simulink model "CMOS_Differential_Stage"
settings: Solver=ode23t  StopTime=0.005  MaxStep=1e-6  RelTol=1e-5  AbsTol=1e-6
undefined symbols (not defined in the file or in its folder): CMOSParams
libraries: fl_lib x18, nesl_utility x9, simulink x2
settings Model: Creator=Final Year B.Tech ECE Project Team  LastModifiedBy=Antigravity MATLAB Automation

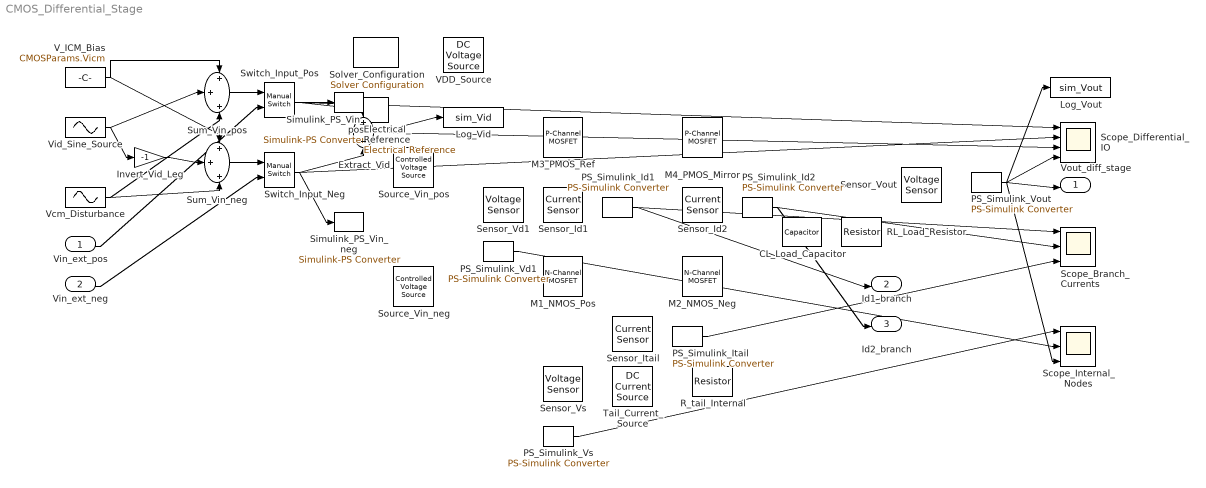
== system CMOS_Differential_Stage ==
  V_ICM_Bias : Constant  Value=CMOSParams.Vicm
  Vid_Sine_Source : Sin  Amplitude=CMOSParams.trans_Vid_peak / 2  Frequency=2*pi*CMOSParams.trans_freq
  Invert_Vid_Leg : Gain  Gain=-1
  Vcm_Disturbance : Sin  Amplitude=CMOSParams.cm_test_amp  Frequency=2*pi*CMOSParams.cm_test_freq
  Sum_Vin_pos : Sum  Inputs=+++
  Sum_Vin_neg : Sum  Inputs=+++
  Vin_ext_pos : Inport  Port=1
  Vin_ext_neg : Inport  Port=2
  Switch_Input_Pos : simulink/Signal Routing/Manual Switch
  Switch_Input_Neg : simulink/Signal Routing/Manual Switch
  Solver_Configuration : nesl_utility/Solver Configuration
  Electrical_Reference : fl_lib/Electrical/Electrical Elements/Electrical Reference
  VDD_Source : fl_lib/Electrical/Electrical Sources/DC Voltage Source  v0=CMOSParams.Vdd
  Simulink_PS_Vin_pos : nesl_utility/Simulink-PS Converter
  Source_Vin_pos : fl_lib/Electrical/Electrical Sources/Controlled Voltage Source
  Simulink_PS_Vin_neg : nesl_utility/Simulink-PS Converter
  Source_Vin_neg : fl_lib/Electrical/Electrical Sources/Controlled Voltage Source
  M1_NMOS_Pos : fl_lib/Electrical/Electrical Elements/N-Channel MOSFET  vth=CMOSParams.nmos.Vth  kp=CMOSParams.nmos.Kp  lambda=CMOSParams.nmos.lambda  rd=CMOSParams.nmos.rd  rs=CMOSParams.nmos.rs
  M2_NMOS_Neg : fl_lib/Electrical/Electrical Elements/N-Channel MOSFET  vth=CMOSParams.nmos.Vth  kp=CMOSParams.nmos.Kp  lambda=CMOSParams.nmos.lambda  rd=CMOSParams.nmos.rd  rs=CMOSParams.nmos.rs
  M3_PMOS_Ref : fl_lib/Electrical/Electrical Elements/P-Channel MOSFET  vth=CMOSParams.pmos.Vth_mag  kp=CMOSParams.pmos.Kp  lambda=CMOSParams.pmos.lambda  rd=CMOSParams.pmos.rd  rs=CMOSParams.pmos.rs
  M4_PMOS_Mirror : fl_lib/Electrical/Electrical Elements/P-Channel MOSFET  vth=CMOSParams.pmos.Vth_mag  kp=CMOSParams.pmos.Kp  lambda=CMOSParams.pmos.lambda  rd=CMOSParams.pmos.rd  rs=CMOSParams.pmos.rs
  Tail_Current_Source : fl_lib/Electrical/Electrical Sources/DC Current Source  i0=CMOSParams.Itail
  R_tail_Internal : fl_lib/Electrical/Electrical Elements/Resistor  R=CMOSParams.Rtail
  CL_Load_Capacitor : fl_lib/Electrical/Electrical Elements/Capacitor  c=CMOSParams.CL
  RL_Load_Resistor : fl_lib/Electrical/Electrical Elements/Resistor  R=CMOSParams.RL
  Sensor_Vout : fl_lib/Electrical/Electrical Sensors/Voltage Sensor
  Sensor_Vd1 : fl_lib/Electrical/Electrical Sensors/Voltage Sensor
  Sensor_Vs : fl_lib/Electrical/Electrical Sensors/Voltage Sensor
  Sensor_Id1 : fl_lib/Electrical/Electrical Sensors/Current Sensor
  Sensor_Id2 : fl_lib/Electrical/Electrical Sensors/Current Sensor
  Sensor_Itail : fl_lib/Electrical/Electrical Sensors/Current Sensor
  PS_Simulink_Vout : nesl_utility/PS-Simulink Converter
  PS_Simulink_Vd1 : nesl_utility/PS-Simulink Converter
  PS_Simulink_Vs : nesl_utility/PS-Simulink Converter
  PS_Simulink_Id1 : nesl_utility/PS-Simulink Converter
  PS_Simulink_Id2 : nesl_utility/PS-Simulink Converter
  PS_Simulink_Itail : nesl_utility/PS-Simulink Converter
  Extract_Vid : Sum  Inputs=+-
  Scope_Differential_IO : Scope  NumInputPorts=4
  Scope_Branch_Currents : Scope  NumInputPorts=3
  Scope_Internal_Nodes : Scope  NumInputPorts=3
  Vout_diff_stage : Outport  Port=1
  Id1_branch : Outport  Port=2
  Id2_branch : Outport  Port=3
  Log_Vout : ToWorkspace  VariableName=sim_Vout  SaveFormat=Structure With Time
  Log_Vid : ToWorkspace  VariableName=sim_Vid  SaveFormat=Structure With Time
  wires:
  V_ICM_Bias/1 -> Sum_Vin_pos/1
  V_ICM_Bias/1 -> Sum_Vin_neg/1
  Vid_Sine_Source/1 -> Sum_Vin_pos/2
  Vid_Sine_Source/1 -> Invert_Vid_Leg/1
  Invert_Vid_Leg/1 -> Sum_Vin_neg/2
  Vcm_Disturbance/1 -> Sum_Vin_pos/3
  Vcm_Disturbance/1 -> Sum_Vin_neg/3
  Sum_Vin_pos/1 -> Switch_Input_Pos/1
  Vin_ext_pos/1 -> Switch_Input_Pos/2
  Sum_Vin_neg/1 -> Switch_Input_Neg/1
  Vin_ext_neg/1 -> Switch_Input_Neg/2
  Switch_Input_Pos/1 -> Simulink_PS_Vin_pos/1
  Switch_Input_Pos/1 -> Extract_Vid/1
  Switch_Input_Pos/1 -> Scope_Differential_IO/1
  Switch_Input_Neg/1 -> Simulink_PS_Vin_neg/1
  Switch_Input_Neg/1 -> Extract_Vid/2
  Switch_Input_Neg/1 -> Scope_Differential_IO/2
  Extract_Vid/1 -> Scope_Differential_IO/3
  Extract_Vid/1 -> Log_Vid/1
  PS_Simulink_Vout/1 -> Scope_Differential_IO/4
  PS_Simulink_Vout/1 -> Scope_Internal_Nodes/3
  PS_Simulink_Vout/1 -> Vout_diff_stage/1
  PS_Simulink_Vout/1 -> Log_Vout/1
  PS_Simulink_Id1/1 -> Scope_Branch_Currents/1
  PS_Simulink_Id1/1 -> Id1_branch/1
  PS_Simulink_Id2/1 -> Scope_Branch_Currents/2
  PS_Simulink_Id2/1 -> Id2_branch/1
  PS_Simulink_Itail/1 -> Scope_Branch_Currents/3
  PS_Simulink_Vs/1 -> Scope_Internal_Nodes/1
  PS_Simulink_Vd1/1 -> Scope_Internal_Nodes/2
